simulink model "day06_initial_state"  (R2024a)
settings: Solver=ode45  StartTime=0.0  StopTime=4  RelTol=1e-8  AbsTol=1e-10
undefined symbols (not defined in the file or in its folder): m, t_step
settings Model: Creator=admin  LastModifiedBy=admin

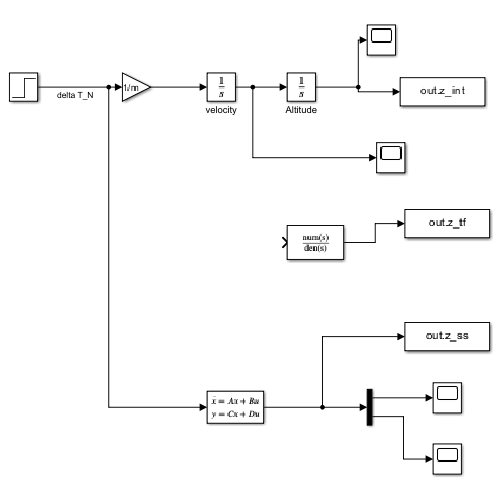
[thumbnail: Simulink's stored preview of the top-level diagram]
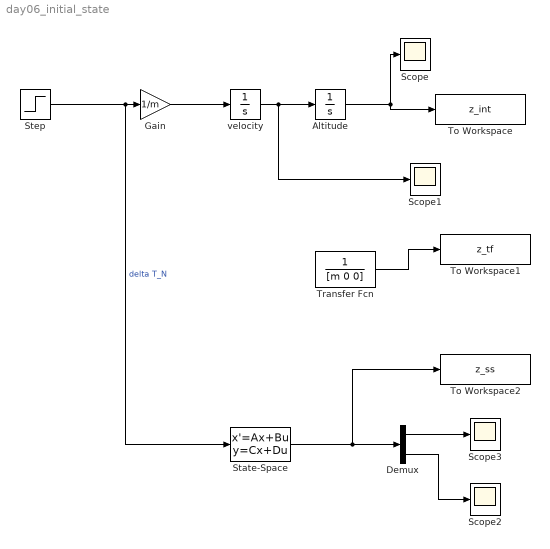
== system day06_initial_state ==
  Altitude : Integrator  InitialCondition=1
  Demux : Demux  Outputs=2
  Gain : Gain  Gain=1/m
  Scope{,1..3} (4 alike) : Scope
  State-Space : StateSpace  A=[0 1;0 0]  B=[0;1/m]  C=[1 0;0 1]  D=[0;0]  InitialCondition=[1;0.3]
  Step : Step  Time=t_step  After=0  SampleTime=0
  To Workspace : ToWorkspace  VariableName=z_int  SaveFormat=Timeseries  SampleTime=-1
  To Workspace1 : ToWorkspace  VariableName=z_tf  SaveFormat=Timeseries  SampleTime=-1
  To Workspace2 : ToWorkspace  VariableName=z_ss  SaveFormat=Timeseries  SampleTime=-1
  Transfer Fcn : TransferFcn  Denominator=[m 0 0]
  velocity : Integrator  InitialCondition=0.3
  wires:
  Gain/1 -> velocity/1
  velocity/1 -> Scope1/1, Altitude/1
  Altitude/1 -> To Workspace/1, Scope/1
  Transfer Fcn/1 -> To Workspace1/1
  Step/1 -> State-Space/1, Gain/1  "delta T_N"
  State-Space/1 -> To Workspace2/1, Demux/1
  Demux/1 -> Scope3/1
  Demux/2 -> Scope2/1
